simulink model "ACC_FFNN_trainbfg_30_30_30_Nor_Sat_Jan_24_RepFast"  (R2021a)
settings: Solver=FixedStepAuto  StartTime=0.0  StopTime=T  RelTol=1e-3
InitFcn:
  | seed = randi(10000);
StartFcn:
  | seed = randi(10000);
undefined symbols (not defined in the file): amax_ego, amin_ego, patch_sig, safe_patch_sig, sw, t_gap, Ts, v0_ego, v0_lead, v_set, x0_ego, x0_lead, x_gain, x_offset, y_gain, y_offset
libraries: neural x95, simulink x3
(part 5 of 5)

== system ACC_FFNN_trainbfg_30_30_30_Nor_Sat_Jan_24_RepFast/Feed-Forward Neural Network/Layer 4/Delays 1 ==
  "p{4}" : Inport  PortDimensions=30
      mask Display: e = 0.06;c1 = [120 230 180]/255;c2 = ([120 230 180]+0)/(256+128);c3 = ([120 230 180]+128)/(256+128);patch([0 1 1 0],[0 0 1 1],c1);patch([0 1 1 1-e 1-e 0+e],[0 0 1 1-e 0+e 0+e],c2);patch([0 0 1 1-e 0+e 0+e],[0 1 1 1-e 1-e 0+e],c3);plot([0 1 1 0 0],[0 0 1 1 0]);
  mux : Mux  Inputs=1
      mask Display: e = 0.06;c1 = [120 150 230]/255;c2 = ([120 150 230]+0)/383;c3 = ([120 150 230]+128)/383;patch([0 1 1 0],[0 0 1 1],c1);patch([0 1 1 1-e 1-e 0+e],[0 0 1 1-e 0+e 0+e],c2);patch([0 0 1 1-e 0+e 0+e],[0 1 1 1-e 1-e 0+e],c3);plot([0 1 1 0 0],[0 0 1 1 0]);disp('Mux')
  "pd{4,3}" : Outport
      mask Display: e = 0.06;c1 = [120 230 180]/255;c2 = ([120 230 180]+0)/(256+128);c3 = ([120 230 180]+128)/(256+128);patch([0 1 1 0],[0 0 1 1],c1);patch([0 1 1 1-e 1-e 0+e],[0 0 1 1-e 0+e 0+e],c2);patch([0 0 1 1-e 0+e 0+e],[0 1 1 1-e 1-e 0+e],c3);plot([0 1 1 0 0],[0 0 1 1 0]);
  wires:
  "p{4}"/1 -> mux/1
  mux/1 -> "pd{4,3}"/1

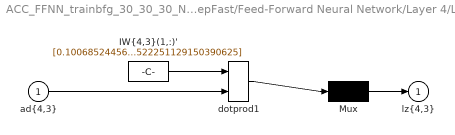
== system ACC_FFNN_trainbfg_30_30_30_Nor_Sat_Jan_24_RepFast/Feed-Forward Neural Network/Layer 4/LW{4,3} ==
  "ad{4,3}" : Inport  PortDimensions=30
      mask Display: e = 0.06;c1 = [120 230 180]/255;c2 = ([120 230 180]+0)/(256+128);c3 = ([120 230 180]+128)/(256+128);patch([0 1 1 0],[0 0 1 1],c1);patch([0 1 1 1-e 1-e 0+e],[0 0 1 1-e 0+e 0+e],c2);patch([0 0 1 1-e 0+e 0+e],[0 1 1 1-e 1-e 0+e],c3);plot([0 1 1 0 0],[0 0 1 1 0]);
  "IW{4,3}(1,:)'" : Constant  Value=[0.10068524456071603623286137008108198642730712890625;-1.2308542746995920769137455863528884947299957275390625;-0.432514488184122802838516008705482818186283111572265625;-0.88161052452166976944880616429145447909832000732421875;1.047250661522342252141015706001780927181243896484375;1.2494820812166036461121620959602296352386474609375;-0.51695141938455602126367693927022628486156463623046875;0.77151093170681728228288420723401941359043121337890625;0.287148303685997585699141154691460542380809783935546875;0.591209777706395822605145440320484340190887451171875;0.253880164017089626771195298715610988438129425048828125;0.41721424808830420705163533057202585041522979736328125;0.08034263617373370303109680889974697493016719818115234375;-1.52573708502251559337992148357443511486053466796875;0.3838249990653010979002601743559353053569793701171875;-0.07377708274661477771960704785669804550707340240478515625;0.261807438869065600695051898583187721669673919677734375;0.41111179003337383619509637355804443359375;-0.51761859208470040183414084822288714349269866943359375;3.497825600071733820328745423466898500919342041015625;0.82009049532437661156336616841144859790802001953125;0.034920957349397714619687604908904177136719226837158203125;-0.85835925297732329486422031550318934023380279541015625;0.5872256891543063961336201828089542686939239501953125;-0.0211520898494626831409792799831848242320120334625244140625;-0.53623519483627590798135997829376719892024993896484375;-0.5719410471487680336366565825301222503185272216796875;0.2478602544512253924580136299482546746730804443359375;-1.23047421873914952783479748177342116832733154296875;0.300420119974777577454005950130522251129150390625]
      mask Display: e = 0.06;c1 = [120 150 230]/255;c2 = ([120 150 230]+0)/383;c3 = ([120 150 230]+128)/383;patch([0 1 1 0],[0 0 1 1],c1);patch([0 1 1 1-e 1-e 0+e],[0 0 1 1-e 0+e 0+e],c2);patch([0 0 1 1-e 0+e 0+e],[0 1 1 1-e 1-e 0+e],c3);plot([0 1 1 0 0],[0 0 1 1 0]);disp('weights');
  Mux : Mux  Inputs=1
      mask Display: e = 0.06;c1 = [120 150 230]/255;c2 = ([120 150 230]+0)/383;c3 = ([120 150 230]+128)/383;patch([0 1 1 0],[0 0 1 1],c1);patch([0 1 1 1-e 1-e 0+e],[0 0 1 1-e 0+e 0+e],c2);patch([0 0 1 1-e 0+e 0+e],[0 1 1 1-e 1-e 0+e],c3);plot([0 1 1 0 0],[0 0 1 1 0]);disp('Mux');
  dotprod1 : neural/Weight Functions/dotprod
  "lz{4,3}" : Outport
      mask Display: e = 0.06;c1 = [120 230 180]/255;c2 = ([120 230 180]+0)/(256+128);c3 = ([120 230 180]+128)/(256+128);patch([0 1 1 0],[0 0 1 1],c1);patch([0 1 1 1-e 1-e 0+e],[0 0 1 1-e 0+e 0+e],c2);patch([0 0 1 1-e 0+e 0+e],[0 1 1 1-e 1-e 0+e],c3);plot([0 1 1 0 0],[0 0 1 1 0]);
  wires:
  "IW{4,3}(1,:)'"/1 -> dotprod1/1
  "ad{4,3}"/1 -> dotprod1/2
  dotprod1/1 -> Mux/1
  Mux/1 -> "lz{4,3}"/1
